simulink model "sm_amrPioneer3DX_path_follow"  (R2025a)
settings: Solver=ode23t  StartTime=0.0  StopTime=35  RelTol=1e-3  AbsTol=1e-4
PostLoadFcn:
  | waypoints = [0 0; 4 2; 3 7; -3 6];
  | target_vel = 0.5;
  | lookahead_d = 2;
  | max_yaw_rate = 1;
StopFcn:
  | %robotPoses = out.yout{1}.Values.Data;
  | 
  | %figure(99);
  | %plot(waypoints(:,1), waypoints(:,2), 'k-x');
  | %hold all
  | %plot(robotPoses(:,1), robotPoses(:,2));
  | %title('XY Waypoint Tracking');
undefined symbols (not defined in the file or in its folder): X, Y, Z
libraries: sm_lib x100, nesl_utility x11, robotalgslib x1, simulink x1
(part 1 of 3)
CloseFcn:
  | try,close(h1_sm_amrPioneer3DX_path_follow),end
  | clear h1_sm_amrPioneer3DX_path_follow
  | try,close(h2_sm_amrPioneer3DX_path_follow),end
  | clear h2_sm_amrPioneer3DX_path_follow
  | try,close(h3_sm_amrPioneer3DX_path_follow),end
  | clear h3_sm_amrPioneer3DX_path_follow
  | try,close(h4_sm_amrPioneer3DX_path_follow),end
  | clear h4_sm_amrPioneer3DX_path_follow
Description:
  | Differential Drive Robot Following a Path
  | Copyright 2021-2025 The MathWorks, Inc.
settings Model: PacingRate=0.011000  Creator=The MathWorks, Inc.  LastModifiedBy=smiller
settings SolverCC: AlgebraicLoopSolver=TrustRegion
settings DataIOCC: MaxDataPoints=10000  SaveOutput=off  ReturnWorkspaceOutputs=off  SignalLoggingName=logsout_sm_amrPioneer3DX_path_follow
settings OptimizationCC: ReuseModelBlockBuffer=off
settings DebuggingCC: UnconnectedInputMsg=warning  UnconnectedOutputMsg=warning  UnconnectedLineMsg=warning  SymbolicDimsDataTypeCodeGenerationDiagnostic=none
settings ModelReferenceCC: EnableRefExpFcnMdlSchedulingChecks=on
settings RTWCC: GPUComputeCapability=3.5  DLArmComputeVersion=19.05
settings SimscapeCC: SimscapeLogType=all  SimscapeLogSimulationStatistics=on  SimscapeLogName=simlog_sm_amrPioneer3DX_path_follow  SimscapeLogDataHistory=10000.0
settings DiagnosticsConfigSet: SimMechanicsConflictingReferenceFrames=none  SimMechanicsRigidlyBoundBlock=none
settings ExplorerConfigSet: InternalSimMechanicsExplorerSettings="<ExplorerConfiguration><canonicalview>default</canonicalview><AnimationSetting><BasePlaybackSpeed>1.0</BasePlaybackSpeed><PlaybackSpeedFactor>4.0</PlaybackSpeedFactor></AnimationSetting><TilePanel><TileInfo><Tiles Columns=\"2\" Count=\"2\" Rows=\"1\"><Column Weight=\"0.5\"/><Column Weight=\"0.5\"/><Row Weight=\"1\"/><Tile Height=\"1\" Width=\"1\" X=\"0\" Y=\"0\"/><Tile Height=\"1\" Width=\"1\" X=\"1\" Y=\"0\"/></Tiles></TileInfo><SceneInfo><SceneViewer><BGColor><R>1</R><G>1</G><B>1</B></BGColor><Camera><DoPerspective>on</DoPerspective><Position><X>-0.845000000000000084</X><Y>0</Y><Z>0.44900000000000001</Z></Position><Center><X>0.139807753012207936</X><Y>0</Y><Z>0.275351822333069651</Z></Center><Up><X>0.173648177666930359</X><Y>0</Y><Z>0.98480775301220802</Z></Up><ViewLimDist>1</ViewLimDist><YLim>0.466307658154998583</YLim><XLim>0.535867364067622698</XLim></Camera></SceneViewer><SceneViewer><BGColor><R>1</R><G>1</G><B>1</B></BGColor><Camera><DoPerspective>off</DoPerspective><Position><X>0.52473266601562496</X><Y>3.27863929130782239</Y><Z>4.85881988452804414</Z></Position><Center><X>0.52473266601562496</X><Y>3.27863929130782239</Y><Z>0.120798183548071592</Z></Center><Up><X>0</X><Y>1</Y><Z>-0</Z></Up><ViewLimDist>1</ViewLimDist><YLim>3.89199849605560333</YLim><XLim>4.47257285734566512</XLim></Camera></SceneViewer></SceneInfo></TilePanel><MechEditorPanel><Cameras><Camera><Id>Camera1</Id><Value><Name>Track_Rear</Name><NativeCamera><PositionTrackingFeature>Robot.Camera.Reference_Frame_Camera_Rear.R</PositionTrackingFeature><CenterTrackingFeature>Robot.Camera.Reference_Frame_Camera_Rear.R</CenterTrackingFeature><UpVectorTrackingFeature>Robot.Camera.Reference_Frame_Camera_Rear.R</UpVectorTrackingFeature><CenterTrackingOrigin>off</CenterTrackingOrigin><CenterTrackingDirection>+X</CenterTrackingDirection><UpVectorTrackingDirection>+Z</UpVectorTrackingDirection></NativeCamera></Value></Camera><Camera><Id>Camera2</Id><Value><Name>Track_Left</Name><NativeCamera><PositionTrackingFeature>Robot.Camera.Reference_Frame_Camera_Left.R</PositionTrackingFeature><CenterTrackingFeature>Robot.Camera.Reference_Frame_Camera_Left.R</CenterTrackingFeature><UpVectorTrackingFeature>Robot.Camera.Reference_Frame_Camera_Left.R</UpVectorTrackingFeature><CenterTrackingOrigin>off</CenterTrackingOrigin><CenterTrackingDirection>+X</CenterTrackingDirection><UpVectorTrackingDirection>+Z</UpVectorTrackingDirection></NativeCamera></Value></Camera></Cameras><GfxPanelCameraMap><MapElement CameraMLId=\"Camera1\" GfxPanelIndex=\"0\"/></GfxPanelCameraMap><VideoCreator><PlaybackSpeedRatio>1.0</PlaybackSpeedRatio><FrameRate>30</FrameRate><VideoFormat>Motion JPEG AVI</VideoFormat><FrameSize>auto</FrameSize></VideoCreator></MechEditorPanel></ExplorerConfiguration>"

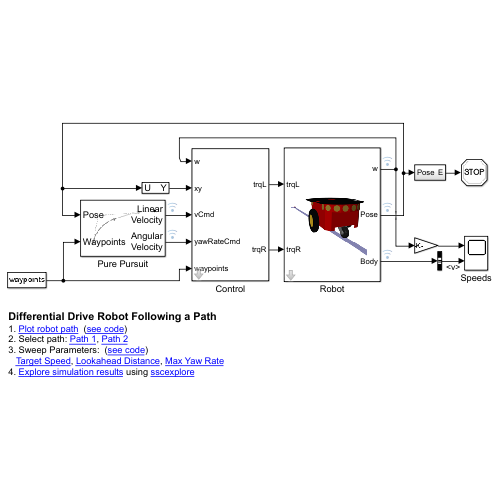
[thumbnail: Simulink's stored preview of the top-level diagram]
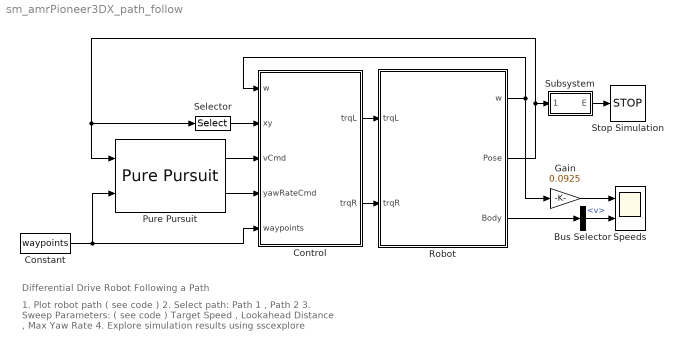
== system sm_amrPioneer3DX_path_follow ==
  note: Differential Drive Robot Following a Path
  note: 1. Plot robot path ( see code )
      | 2. Select path: Path 1 , Path 2
      | 3. Sweep Parameters: ( see code )
      | Target Speed , Lookahead Distance , Max Yaw Rate
      | 4. Explore simulation results using sscexplore
  Bus Selector : BusSelector  OutputSignals=v
  Constant : Constant  Value=waypoints
  Control : Subsystem  mask(Control for Differential Drive Robot){xTrack=0.3, rWheel=0.0925, xSlow=0.5, xStop=0.1, kp=0.8}
      mask prompts: xTrack "Robot Drive Wheel Radius (m)"; rWheel "Robot Track Width (m)"; xSlow "Distance from end to slow (m)"; xStop "Distance from end to stop (m)"; kp "Controller Proportional Gain"
      mask help: Determines torque commands for wheels based on target speed and target yaw rate of robot. As robot approaches final waypoint, speed is ramped down to 0.
  Gain : Gain  Gain=0.0925
  Pure Pursuit : robotalgslib/Pure Pursuit  DesiredLinearVelocityPort=off  DesiredLinearVelocity=target_vel  MaxAngularVelocity=max_yaw_rate  LookaheadDistancePort=off  LookaheadDistance=lookahead_d  TargetDirPort=off  SimulateUsing=Code generation
  Robot : Subsystem  mask(Differential Drive Robot){kWheel=1e4, dWheel=1e3, xtrWheel=1e-3, muk=0.9, mud=0.8, vth=1e-3, checkbox_start=on, waypoint_list=waypoints, init_xy_user=[0 0], init_orient_user=0, clr_contact_sphere=[0 1 0], opc_contact_sphere=0}
      mask prompts: kWheel "Stiffness (N/m)"; dWheel "Damping (N/(m/s))"; xtrWheel "Transition Region Width (m)"; muk "Static Friction Coefficient"; mud "Dynamic Friction Coefficient"; vth "Critical Velocity (m/s)"; checkbox_start "Start at first waypoint"; waypoint_list "Waypoints [xy] (m)"; init_xy_user "Initial Position [x y] (m)"; init_orient_user "Initial Orientation  (0 = +x) (deg)"; clr_contact_sphere "Color Contact Spheres [RGB]"; opc_contact_sphere "Opacity Contact Spheres"
      mask help: Set contact, friction, and initial pose for robot.
      mask init:
      | if (strcmp(get_param(gcb,'checkbox_start'),'on'))
      |   init_orient = atan2(waypoint_list(2,2)-waypoint_list(1,2),waypoint_list(2,1)-waypoint_list(1,1))*180/pi;
      |   init_xy = waypoint_list(1,:);
      | else
      |   init_xy     = init_xy_user;
      |   init_orient = init_orient_user;
      | end
      mask Callback checkbox_start:
      | maskObj = Simulink.Mask.get(gcb);
      | wpl_h = maskObj.getParameter('waypoint_list');
      | ixy_h = maskObj.getParameter('init_xy_user');
      | ior_h = maskObj.getParameter('init_orient_user');
      | if (strcmp(get_param(gcb,'checkbox_start'),'on'))
      |     wpl_h.Visible = 'on';
      |     ixy_h.Visible = 'off';
      |     ior_h.Visible = 'off';
      | else
      |     wpl_h.Visible = 'off';
      |     ixy_h.Visible = 'on';
      |     ior_h.Visible = 'on';
      | end
      mask DialogControl grp_whl_contact Prompt: Wheel Contact
      mask Display: image('sm_amrPioneer3DX_path_follow_robot.png')
  Selector : Selector  InputPortWidth=3  IndexOptions=Index vector (dialog)  Indices=[1 2]  OutputSizes=1
  Speeds : Scope  NumInputPorts=2
      settings: ActiveDisplayYMinimum=-0.11386  ActiveDisplayYMaximum=1.02475
  Stop Simulation : Stop
  Subsystem : Subsystem
  wires:
  Constant/1 -> Pure Pursuit/2, Control/5(waypoints)
  Robot/1(w) -> Gain/1, Control/1(w)
  Robot/2(Pose) -> Selector/1, Pure Pursuit/1, Subsystem/1(Pose)
  Gain/1 -> Speeds/1
  Robot/3(Body) -> Bus Selector/1
  Pure Pursuit/1 -> Control/3(vCmd)
  Pure Pursuit/2 -> Control/4(yawRateCmd)
  Control/1(trqL) -> Robot/1(trqL)
  Control/2(trqR) -> Robot/2(trqR)
  Selector/1 -> Control/2(xy)
  Subsystem/1(E) -> Stop Simulation/1
  Bus Selector/1 -> Speeds/2  "<v>"

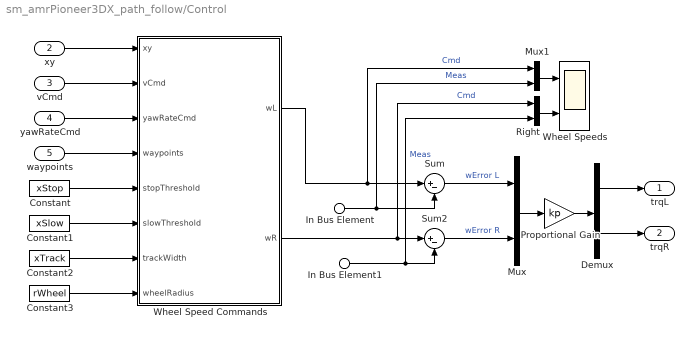
== system sm_amrPioneer3DX_path_follow/Control ==
  In Bus Element : Inport  PortName=w  Element=L
  In Bus Element1 : Inport  PortName=w  Element=R
  xy : Inport  Port=2
  vCmd : Inport  Port=3
  yawRateCmd : Inport  Port=4
  waypoints : Inport  Port=5
  Constant : Constant  Value=xStop
  Constant1 : Constant  Value=xSlow
  Constant2 : Constant  Value=xTrack
  Constant3 : Constant  Value=rWheel
  Demux : Demux  Outputs=2
  Mux : Mux  Inputs=2
  Mux1 : Mux  Inputs=2
  Proportional Gain : Gain  Gain=kp
  Right : Mux  Inputs=2
  Sum : Sum  Inputs=|+-
  Sum2 : Sum  Inputs=|+-
  Wheel Speed Commands : MATLAB Function  TreatAsAtomicUnit=on
  Wheel Speeds : Scope  NumInputPorts=2
      settings: Title=Left Wheel  ActiveDisplayYMinimum=-0.75851  ActiveDisplayYMaximum=6.82662  DataLoggingVariableName=ScopeData2
  trqL : Outport
  trqR : Outport  Port=2
  wires:
  Demux/1 -> trqL/1
  yawRateCmd/1 -> Wheel Speed Commands/3(yawRateCmd)
  xy/1 -> Wheel Speed Commands/1(xy)
  vCmd/1 -> Wheel Speed Commands/2(vCmd)
  Demux/2 -> trqR/1
  waypoints/1 -> Wheel Speed Commands/4(waypoints)
  Constant/1 -> Wheel Speed Commands/5(stopThreshold)
  Constant1/1 -> Wheel Speed Commands/6(slowThreshold)
  Constant2/1 -> Wheel Speed Commands/7(trackWidth)
  Constant3/1 -> Wheel Speed Commands/8(wheelRadius)
  Wheel Speed Commands/1(wL) -> Mux1/1, Sum/1  "Cmd"
  Wheel Speed Commands/2(wR) -> Right/1, Sum2/1  "Cmd"
  Sum2/1 -> Mux/2  "wError R"
  In Bus Element1/1 -> Sum2/2, Right/2  "Meas"
  In Bus Element/1 -> Mux1/2, Sum/2  "Meas"
  Mux/1 -> Proportional Gain/1
  Proportional Gain/1 -> Demux/1
  Sum/1 -> Mux/1  "wError L"
  Mux1/1 -> Wheel Speeds/1
  Right/1 -> Wheel Speeds/2

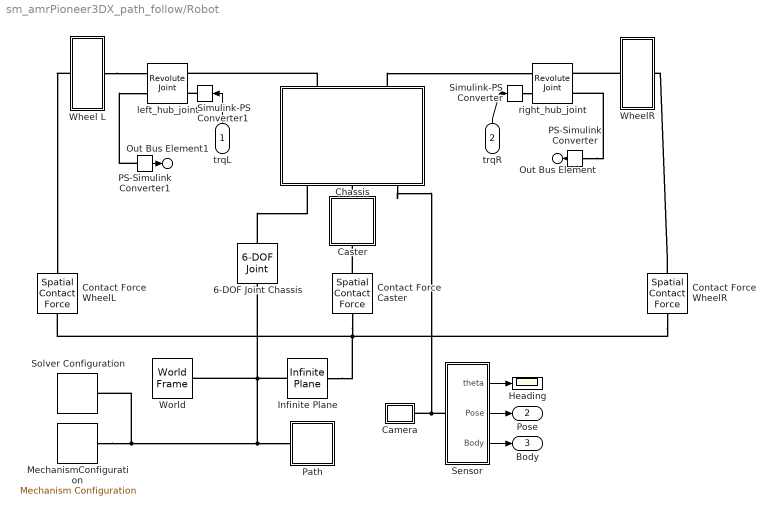
== system sm_amrPioneer3DX_path_follow/Robot ==
  trqL : Inport
  trqR : Inport  Port=2
  6-DOF Joint Chassis : sm_lib/Joints/6-DOF Joint  JointMode=Normal  CompositeWrenchDir=FollowerOnBase  CompositeWrenchFrame=BaseFrame  SenseConstraintForce=off  SenseConstraintTorque=off  SenseTotalForce=off  SenseTotalTorque=off  PxPositionTargetSpecify=on  PxPositionTargetPriority=High  PxPositionTargetValue=init_xy(1)  PxPositionTargetValueUnits=m  PxVelocityTargetSpecify=off  PxVelocityTargetPriority=High  PxVelocityTargetValue=0  PxVelocityTargetValueUnits=m/s  PxEquilibriumPosition=0  PxEquilibriumPositionUnits=m  PxSpringStiffness=0  PxSpringStiffnessUnits=N/m  PxDampingCoefficient=0  PxDampingCoefficientUnits=N/(m/s)  PxLowerLimitSpecify=off  PxLowerLimitBound=-1  PxLowerLimitBoundUnits=m  PxLowerLimitStiffness=1e6  PxLowerLimitStiffnessUnits=N/m  PxLowerLimitDamping=1e3  PxLowerLimitDampingUnits=N/(m/s)  PxLowerLimitTransitionRegionWidth=1e-4  PxLowerLimitTransitionRegionWidthUnits=m  PxUpperLimitSpecify=off  PxUpperLimitBound=1  PxUpperLimitBoundUnits=m  PxUpperLimitStiffness=1e6  PxUpperLimitStiffnessUnits=N/m  PxUpperLimitDamping=1e3  PxUpperLimitDampingUnits=N/(m/s)  PxUpperLimitTransitionRegionWidth=1e-4  PxUpperLimitTransitionRegionWidthUnits=m  PxTorqueActuationMode=NoTorque  PxMotionActuationMode=ComputedMotion  PxSensePosition=off  PxSenseVelocity=off  PxSenseAcceleration=off  PxSenseTorqueForce=off  PxSenseLowerLimitTorqueForce=off  PxSenseUpperLimitTorqueForce=off  PyPositionTargetSpecify=on  PyPositionTargetPriority=High  PyPositionTargetValue=init_xy(2)  PyPositionTargetValueUnits=m  PyVelocityTargetSpecify=off  PyVelocityTargetPriority=High  PyVelocityTargetValue=0  PyVelocityTargetValueUnits=m/s  PyEquilibriumPosition=0  PyEquilibriumPositionUnits=m  PySpringStiffness=0  PySpringStiffnessUnits=N/m  PyDampingCoefficient=0  PyDampingCoefficientUnits=N/(m/s)  PyLowerLimitSpecify=off  PyLowerLimitBound=-1  PyLowerLimitBoundUnits=m  PyLowerLimitStiffness=1e6  PyLowerLimitStiffnessUnits=N/m  PyLowerLimitDamping=1e3  PyLowerLimitDampingUnits=N/(m/s)  PyLowerLimitTransitionRegionWidth=1e-4  PyLowerLimitTransitionRegionWidthUnits=m  PyUpperLimitSpecify=off  PyUpperLimitBound=1  PyUpperLimitBoundUnits=m  PyUpperLimitStiffness=1e6  PyUpperLimitStiffnessUnits=N/m  PyUpperLimitDamping=1e3  PyUpperLimitDampingUnits=N/(m/s)  PyUpperLimitTransitionRegionWidth=1e-4  PyUpperLimitTransitionRegionWidthUnits=m  PyTorqueActuationMode=NoTorque  PyMotionActuationMode=ComputedMotion  PySensePosition=off  PySenseVelocity=off  PySenseAcceleration=off  PySenseTorqueForce=off  PySenseLowerLimitTorqueForce=off  PySenseUpperLimitTorqueForce=off  PzPositionTargetSpecify=on  PzPositionTargetPriority=High  PzPositionTargetValue=0.015  PzPositionTargetValueUnits=m  PzVelocityTargetSpecify=off  PzVelocityTargetPriority=High  PzVelocityTargetValue=0  PzVelocityTargetValueUnits=m/s  PzEquilibriumPosition=0  PzEquilibriumPositionUnits=m  PzSpringStiffness=0  PzSpringStiffnessUnits=N/m  PzDampingCoefficient=0  PzDampingCoefficientUnits=N/(m/s)  PzLowerLimitSpecify=off  PzLowerLimitBound=-1  PzLowerLimitBoundUnits=m  PzLowerLimitStiffness=1e6  PzLowerLimitStiffnessUnits=N/m  PzLowerLimitDamping=1e3  PzLowerLimitDampingUnits=N/(m/s)  PzLowerLimitTransitionRegionWidth=1e-4  PzLowerLimitTransitionRegionWidthUnits=m  PzUpperLimitSpecify=off  PzUpperLimitBound=1  PzUpperLimitBoundUnits=m  PzUpperLimitStiffness=1e6  PzUpperLimitStiffnessUnits=N/m  PzUpperLimitDamping=1e3  PzUpperLimitDampingUnits=N/(m/s)  PzUpperLimitTransitionRegionWidth=1e-4  PzUpperLimitTransitionRegionWidthUnits=m  PzTorqueActuationMode=NoTorque  PzMotionActuationMode=ComputedMotion  PzSensePosition=off  PzSenseVelocity=off  PzSenseAcceleration=off  PzSenseTorqueForce=off  PzSenseLowerLimitTorqueForce=off  PzSenseUpperLimitTorqueForce=off  SphPositionTargetSpecify=on  SphPositionTargetPriority=High  SphPositionTargetRotationMethod=StandardAxis  SphPositionTargetFollAlignAxisA=+X  SphPositionTargetBaseAlignAxisA=+Y  SphPositionTargetFollAlignAxisB=+Y  SphPositionTargetBaseAlignAxisB=+Z  SphPositionTargetRotationStandardAxis=+Z  SphPositionTargetRotationAngle=init_orient  SphPositionTargetRotationAngleUnits=deg  SphPositionTargetRotationArbitraryAxis=[0 0 1]  SphPositionTargetRotationSequenceAxes=FollowerAxes  SphPositionTargetRotationSequence=XYX  SphPositionTargetRotationSequenceAngles=[0 0 0]  SphPositionTargetRotationSequenceAnglesUnits=deg  SphPositionTargetRotationMatrix=[1 0 0; 0 1 0; 0 0 1]  SphPositionTargetQuaternion=[1 0 0 0]  SphVelocityTargetSpecify=off  SphVelocityTargetPriority=High  SphVelocityTargetValue=[0 0 0]  SphVelocityTargetValueUnits=deg/s  SphVelocityTargetInFollowerFrame=on  SphEqPosRotationMethod=None  SphEqPosFollAlignAxisA=+X  SphEqPosBaseAlignAxisA=+Y  SphEqPosFollAlignAxisB=+Y  SphEqPosBaseAlignAxisB=+Z  SphEqPosRotationStandardAxis=+Z  SphEqPosRotationAngle=0.0  SphEqPosRotationAngleUnits=deg  SphEqPosRotationArbitraryAxis=[0 0 1]  SphEqPosRotationSequenceAxes=FollowerAxes  SphEqPosRotationSequence=XYX  SphEqPosRotationSequenceAngles=[0 0 0]  SphEqPosRotationSequenceAnglesUnits=deg  SphEqPosRotationMatrix=[1 0 0; 0 1 0; 0 0 1]  SphEqPosQuaternion=[1 0 0 0]  SphSpringStiffness=0  SphSpringStiffnessUnits=N*m/deg  SphDampingCoefficient=0  SphDampingCoefficientUnits=N*m/(deg/s)  SphLowerLimitSpecify=off  SphLowerLimitBound=15  SphLowerLimitBoundUnits=deg  SphLowerLimitStiffness=1e4  SphLowerLimitStiffnessUnits=N*m/deg  SphLowerLimitDamping=10  SphLowerLimitDampingUnits=N*m/(deg/s)  SphLowerLimitTransitionRegionWidth=0.1  SphLowerLimitTransitionRegionWidthUnits=deg  SphUpperLimitSpecify=off  SphUpperLimitBound=45  SphUpperLimitBoundUnits=deg  SphUpperLimitStiffness=1e4  SphUpperLimitStiffnessUnits=N*m/deg  SphUpperLimitDamping=10  SphUpperLimitDampingUnits=N*m/(deg/s)  SphUpperLimitTransitionRegionWidth=0.1  SphUpperLimitTransitionRegionWidthUnits=deg  SphTorqueActuationMode=NoTorque  SphActuateTorqueX=off  SphActuateTorqueY=off  SphActuateTorqueZ=off  SphActuateTorque=off  SphActuationFrame=BaseFrame  SphSensePosition=off  SphSenseVelocityX=off  SphSenseVelocityY=off  SphSenseVelocityZ=off  SphSenseVelocity=off  SphSenseAccelerationX=off  SphSenseAccelerationY=off  SphSenseAccelerationZ=off  SphSenseAcceleration=off  SphSenseLowerLimitTorqueMag=off  SphSenseUpperLimitTorqueMag=off  SphSensingFrame=BaseFrame
  Camera : Subsystem
  Caster : Subsystem
  Chassis : Subsystem
  Contact Force Caster : sm_lib/Forces and Torques/Spatial Contact Force  SenseSeparationDistance=off  NormalForceType=SmoothSpringDamper  NormalStiffness=kWheel  NormalStiffnessUnits=N/m  NormalDamping=dWheel  NormalDampingUnits=N/(m/s)  NormalTransitionRegionWidth=xtrWheel  NormalTransitionRegionWidthUnits=m  FrictionType=SmoothStickSlip  CoefficientOfStaticFriction=muk  CoefficientOfDynamicFriction=mud  FrictionalCriticalVelocity=vth  FrictionalCriticalVelocityUnits=m/s  SenseContactSignal=off  SensePenetrationDepth=off  SenseNormalVelocity=off  SenseTangentialVelocity=off  SensingForceTorqueDirection=BaseOnFollower  SensingForceTorqueResolutionFrame=ContactFrame  SenseNormalForce=off  SenseNormalForceMagnitude=off  SenseNormalTorque=off  SenseFrictionalForce=off  SenseFrictionalForceMagnitude=off  SenseFrictionalTorque=off  SenseTotalForce=off  SenseTotalTorque=off  SenseContactBaseRotation=off  SenseContactBaseTranslation=off  SenseContactFollowerRotation=off  SenseContactFollowerTranslation=off  ZeroCrossDetectContactStartAndEnd=off
  Contact Force WheelL : sm_lib/Forces and Torques/Spatial Contact Force  SenseSeparationDistance=off  NormalForceType=SmoothSpringDamper  NormalStiffness=kWheel  NormalStiffnessUnits=N/m  NormalDamping=dWheel  NormalDampingUnits=N/(m/s)  NormalTransitionRegionWidth=xtrWheel  NormalTransitionRegionWidthUnits=m  FrictionType=SmoothStickSlip  CoefficientOfStaticFriction=muk  CoefficientOfDynamicFriction=mud  FrictionalCriticalVelocity=vth  FrictionalCriticalVelocityUnits=m/s  SenseContactSignal=off  SensePenetrationDepth=off  SenseNormalVelocity=off  SenseTangentialVelocity=off  SensingForceTorqueDirection=BaseOnFollower  SensingForceTorqueResolutionFrame=ContactFrame  SenseNormalForce=off  SenseNormalForceMagnitude=off  SenseNormalTorque=off  SenseFrictionalForce=off  SenseFrictionalForceMagnitude=off  SenseFrictionalTorque=off  SenseTotalForce=off  SenseTotalTorque=off  SenseContactBaseRotation=off  SenseContactBaseTranslation=off  SenseContactFollowerRotation=off  SenseContactFollowerTranslation=off  ZeroCrossDetectContactStartAndEnd=off
  Contact Force WheelR : sm_lib/Forces and Torques/Spatial Contact Force  SenseSeparationDistance=off  NormalForceType=SmoothSpringDamper  NormalStiffness=kWheel  NormalStiffnessUnits=N/m  NormalDamping=dWheel  NormalDampingUnits=N/(m/s)  NormalTransitionRegionWidth=xtrWheel  NormalTransitionRegionWidthUnits=m  FrictionType=SmoothStickSlip  CoefficientOfStaticFriction=muk  CoefficientOfDynamicFriction=mud  FrictionalCriticalVelocity=vth  FrictionalCriticalVelocityUnits=m/s  SenseContactSignal=off  SensePenetrationDepth=off  SenseNormalVelocity=off  SenseTangentialVelocity=off  SensingForceTorqueDirection=BaseOnFollower  SensingForceTorqueResolutionFrame=ContactFrame  SenseNormalForce=off  SenseNormalForceMagnitude=off  SenseNormalTorque=off  SenseFrictionalForce=off  SenseFrictionalForceMagnitude=off  SenseFrictionalTorque=off  SenseTotalForce=off  SenseTotalTorque=off  SenseContactBaseRotation=off  SenseContactBaseTranslation=off  SenseContactFollowerRotation=off  SenseContactFollowerTranslation=off  ZeroCrossDetectContactStartAndEnd=off
  Heading : Scope
      settings: ActiveDisplayYMinimum=-3.92553  ActiveDisplayYMaximum=3.92324
  Infinite Plane : sm_lib/Curves and Surfaces/Infinite Plane  GraphicType=Rectangle  GraphicPlaneWidth=1  GraphicPlaneWidthUnits=m  GraphicPlaneHeight=1  GraphicPlaneHeightUnits=m  GraphicVisPropType=SimpleVisualProperties  GraphicDiffuseColor=[0.5 0.5 0.5]  GraphicOpacity=0.25  GraphicSpecularColor=[0.5 0.5 0.5 1.0]  GraphicAmbientColor=[0.15 0.15 0.15 1.0]  GraphicEmissiveColor=[0.0 0.0 0.0 1.0]  GraphicShininess=75
  MechanismConfiguration : sm_lib/Utilities/Mechanism Configuration  UniformGravity=Constant  GravityVector=[0 0 -9.80665]  GravityVectorUnits=m/s^2  LinearizationDelta=0.001  JointModeTransitionNonlinearIterations=2
  PS-Simulink Converter : nesl_utility/PS-Simulink Converter  PhysicalDomain=network_engine_domain  SubClassName=ps_output  LeftPortType=input  RightPortType=output  PseudoPeriodic=off  Frequencies=[]  VectorFormat=1-D array  Unit=inherit  AffineConversion=off
  PS-Simulink Converter1 : nesl_utility/PS-Simulink Converter  PhysicalDomain=network_engine_domain  SubClassName=ps_output  LeftPortType=input  RightPortType=output  PseudoPeriodic=off  Frequencies=[]  VectorFormat=1-D array  Unit=inherit  AffineConversion=off
  Path : Subsystem  mask(Visualize Path of Waypoints){waypoints=waypoints, path_width=0.03, path_depth=0.01, clr_path=[0.6 0.6 1], opc_path=0.5, pt_rad=2e-2, pt_clr=[0.6353 0.07843 0.1843], pt_opc=0.8}
      mask prompts: waypoints "Waypoints [x y] (m)"; path_width "Path Width (m)"; path_depth "Path Depth (m)"; clr_path "Path Color [RGB]"; opc_path "Path Opacity (0-1)"; pt_rad "Waypoints Radius"; pt_clr "Waypoints Color [RGB]"; pt_opc "Waypoints Opacity (0-1)"
      mask help: Visualize path of waypoints using point cloud for points and extrusion for path. Path must not cross itself.
      mask init:
      | xy_data = Extr_Data_Waypoints(waypoints,path_width);
  Sensor : Subsystem
  Simulink-PS Converter : nesl_utility/Simulink-PS Converter  PhysicalDomain=network_engine_domain  SubClassName=ps_input  LeftPortType=input  RightPortType=output  PseudoPeriodic=off  Frequencies=[]  NoiseDistribution=none  NoiseParameters=[]  Unit=1  AffineConversion=off  FilteringAndDerivatives=provide  SimscapeFilterOrder=1  InputFilterTimeConstant=0.001  UdotUserProvided=0
  Simulink-PS Converter1 : nesl_utility/Simulink-PS Converter  PhysicalDomain=network_engine_domain  SubClassName=ps_input  LeftPortType=input  RightPortType=output  PseudoPeriodic=off  Frequencies=[]  NoiseDistribution=none  NoiseParameters=[]  Unit=1  AffineConversion=off  FilteringAndDerivatives=provide  SimscapeFilterOrder=1  InputFilterTimeConstant=0.001  UdotUserProvided=0
  Solver Configuration : nesl_utility/Solver Configuration  PhysicalDomain=network_engine_domain  SubClassName=solver  LeftPortType=input  RightPortType=generic  Tones=[]  Harmonics=[]  SimulateNoise=off  Profile=off  UseLocalSampling=off  EnableSwitchedLinearOptims=on  FrequencyDomain=off  UseCCode=off  RelTol=0.001  AbsTol=1e-06  MinStep=1e-09  ToWorkspace=off  RevertToSquareIcSolve=off  NumHomotopyIterations=100  PhasorMode=off  PhasorModeNumHarmonics=1  ConsistencySolver=NEWTON_FTOL  IndexReductionMethod=DerivativeReplacement  DoDC=off  ResidualTolerance=1e-09  ConsistencyTolSource=GLOBAL  ConsistencyAbsTol=0.001  ConsistencyRelTol=0.001  ConsistencyTolFactor=0.001  UseLocalSolver=off  LocalSolverChoice=NE_BACKWARD_EULER_ADVANCER  ResolveIndetEquations=on  FunctionEvalNumThread=1  LocalSolverSampleTime=0.001  DoFixedCost=off  MaxNonlinIter=3  MaxModeIter=2  ComputeImpulses=off  ImpulseIterations=2  LinearAlgebra=auto  LinearAlgebraNumThread=0  EquationFormulation=NE_TIME_EF  DelaysMemoryBudget=1024  AutomaticFiltering=on  FilteringTimeConstant=0.001  PartitionStorageMethod=AS_NEEDED  PartitionMemoryBudget=1024  PartitionMethod=ROBUST  MultibodyUseLocalSolver=off  MultibodyLocalSolverChoice=ODE1  MultibodyLocalSolverSampleTime=0.001
  Wheel L : Subsystem
  WheelR : Subsystem
  World : sm_lib/Frames and Transforms/World Frame
  left_hub_joint : sm_lib/Joints/Revolute Joint  JointMode=Normal  CompositeWrenchDir=FollowerOnBase  CompositeWrenchFrame=BaseFrame  SenseConstraintForce=off  SenseConstraintTorque=off  SenseTotalForce=off  SenseTotalTorque=off  PositionTargetSpecify=off  PositionTargetPriority=High  PositionTargetValue=0  PositionTargetValueUnits=deg  VelocityTargetSpecify=off  VelocityTargetPriority=High  VelocityTargetValue=0  VelocityTargetValueUnits=deg/s  EquilibriumPosition=0  EquilibriumPositionUnits=deg  SpringStiffness=0  SpringStiffnessUnits=N*m/deg  DampingCoefficient=0  DampingCoefficientUnits=m^2*kg/s/rad  LowerLimitSpecify=off  LowerLimitBound=-90  LowerLimitBoundUnits=deg  LowerLimitStiffness=1e4  LowerLimitStiffnessUnits=N*m/deg  LowerLimitDamping=10  LowerLimitDampingUnits=N*m/(deg/s)  LowerLimitTransitionRegionWidth=0.1  LowerLimitTransitionRegionWidthUnits=deg  UpperLimitSpecify=off  UpperLimitBound=90  UpperLimitBoundUnits=deg  UpperLimitStiffness=1e4  UpperLimitStiffnessUnits=N*m/deg  UpperLimitDamping=10  UpperLimitDampingUnits=N*m/(deg/s)  UpperLimitTransitionRegionWidth=0.1  UpperLimitTransitionRegionWidthUnits=deg  TorqueActuationMode=InputTorque  MotionActuationMode=ComputedMotion  SensePosition=off  SenseVelocity=on  SenseAcceleration=off  SenseTorqueForce=off  SenseLowerLimitTorqueForce=off  SenseUpperLimitTorqueForce=off
  right_hub_joint : sm_lib/Joints/Revolute Joint  JointMode=Normal  CompositeWrenchDir=FollowerOnBase  CompositeWrenchFrame=BaseFrame  SenseConstraintForce=off  SenseConstraintTorque=off  SenseTotalForce=off  SenseTotalTorque=off  PositionTargetSpecify=off  PositionTargetPriority=High  PositionTargetValue=0  PositionTargetValueUnits=deg  VelocityTargetSpecify=off  VelocityTargetPriority=High  VelocityTargetValue=0  VelocityTargetValueUnits=deg/s  EquilibriumPosition=0  EquilibriumPositionUnits=deg  SpringStiffness=0  SpringStiffnessUnits=N*m/deg  DampingCoefficient=0  DampingCoefficientUnits=m^2*kg/s/rad  LowerLimitSpecify=off  LowerLimitBound=-90  LowerLimitBoundUnits=deg  LowerLimitStiffness=1e4  LowerLimitStiffnessUnits=N*m/deg  LowerLimitDamping=10  LowerLimitDampingUnits=N*m/(deg/s)  LowerLimitTransitionRegionWidth=0.1  LowerLimitTransitionRegionWidthUnits=deg  UpperLimitSpecify=off  UpperLimitBound=90  UpperLimitBoundUnits=deg  UpperLimitStiffness=1e4  UpperLimitStiffnessUnits=N*m/deg  UpperLimitDamping=10  UpperLimitDampingUnits=N*m/(deg/s)  UpperLimitTransitionRegionWidth=0.1  UpperLimitTransitionRegionWidthUnits=deg  TorqueActuationMode=InputTorque  MotionActuationMode=ComputedMotion  SensePosition=off  SenseVelocity=on  SenseAcceleration=off  SenseTorqueForce=off  SenseLowerLimitTorqueForce=off  SenseUpperLimitTorqueForce=off
  Out Bus Element : Outport  PortName=w  Element=R
  Out Bus Element1 : Outport  PortName=w  Element=L
  Pose : Outport  Port=2
  Body : Outport  Port=3
  wires:
  PS-Simulink Converter1/1 -> Out Bus Element1/1
  PS-Simulink Converter/1 -> Out Bus Element/1
  trqR/1 -> Simulink-PS Converter/1
  trqL/1 -> Simulink-PS Converter1/1
  Sensor/3(Body) -> Body/1
  Sensor/1(theta) -> Heading/1
  Sensor/2(Pose) -> Pose/1
  connections:
  Infinite Plane/RConn1 -- Contact Force WheelR/LConn1 -- Contact Force Caster/LConn1 -- Contact Force WheelL/LConn1
  MechanismConfiguration/RConn1 -- Solver Configuration/RConn1 -- World/RConn1 -- Infinite Plane/LConn1 -- 6-DOF Joint Chassis/LConn1 -- Path/LConn1
  Simulink-PS Converter1/RConn1 -- left_hub_joint/LConn2
  PS-Simulink Converter/LConn1 -- right_hub_joint/RConn2
  PS-Simulink Converter1/LConn1 -- left_hub_joint/RConn2
  Simulink-PS Converter/RConn1 -- right_hub_joint/LConn2
  Chassis/RConn2 -- right_hub_joint/LConn1
  Chassis/RConn1 -- left_hub_joint/LConn1
  6-DOF Joint Chassis/RConn1 -- Chassis/LConn1
  Caster/LConn1 -- Chassis/LConn2
  Contact Force Caster/RConn1 -- Caster/RConn1
  WheelR/LConn1 -- right_hub_joint/RConn1
  Contact Force WheelR/RConn1 -- WheelR/RConn1
  Wheel L/RConn1 -- left_hub_joint/RConn1
  Wheel L/LConn1 -- Contact Force WheelL/RConn1
  Sensor/LConn1 -- Chassis/LConn3 -- Camera/LConn1

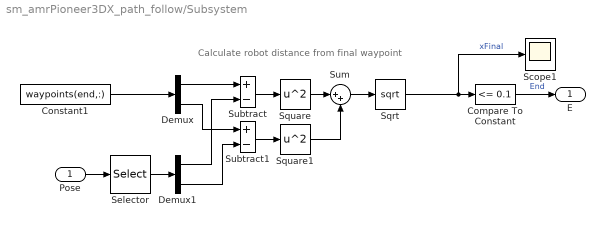
== system sm_amrPioneer3DX_path_follow/Subsystem ==
  note: Calculate robot distance
      | from final waypoint
  Pose : Inport
  Compare To Constant : simulink/Logic and Bit Operations/Compare To Constant  relop=<=  const=0.1  OutDataTypeStr=boolean
  Constant1 : Constant  Value=waypoints(end,:)
  Demux : Demux  Outputs=2
  Demux1 : Demux  Outputs=2
  Scope1 : Scope
      settings: ActiveDisplayYMinimum=-0.84679  ActiveDisplayYMaximum=8.62109  DataLoggingVariableName=ScopeData2
  Selector : Selector  InputPortWidth=3  IndexOptions=Index vector (dialog)  Indices=[1 2]  OutputSizes=1
  Sqrt : Sqrt
  Square : Math  Operator=square
  Square1 : Math  Operator=square
  Subtract : Sum  Inputs=+-
  Subtract1 : Sum  Inputs=+-
  Sum : Sum  Inputs=|++
  E : Outport
  wires:
  Constant1/1 -> Demux/1
  Pose/1 -> Selector/1
  Demux/1 -> Subtract/1
  Selector/1 -> Demux1/1
  Demux1/1 -> Subtract/2
  Demux/2 -> Subtract1/1
  Demux1/2 -> Subtract1/2
  Subtract/1 -> Square/1
  Subtract1/1 -> Square1/1
  Square/1 -> Sum/1
  Square1/1 -> Sum/2
  Sum/1 -> Sqrt/1
  Sqrt/1 -> Compare To Constant/1, Scope1/1  "xFinal"
  Compare To Constant/1 -> E/1  "End"

== system sm_amrPioneer3DX_path_follow/Robot/Camera ==
  Reference Frame Camera Left : sm_lib/Frames and Transforms/Reference Frame
  Reference Frame Camera Rear : sm_lib/Frames and Transforms/Reference Frame
  Transform Camera Left : sm_lib/Frames and Transforms/Rigid Transform  RotationMethod=RotationSequence  FollAlignAxisA=+X  BaseAlignAxisA=+Y  FollAlignAxisB=+Y  BaseAlignAxisB=+Z  RotationStandardAxis=+Y  RotationAngle=10  RotationAngleUnits=deg  RotationArbitraryAxis=[0 0 1]  RotationSequenceAxes=FollowerAxes  RotationSequence=ZYX  RotationSequenceAngles=[-90 10 0]  RotationSequenceAnglesUnits=deg  RotationMatrix=[1 0 0; 0 1 0; 0 0 1]  Quaternion=[1 0 0 0]  TranslationMethod=Cartesian  TranslationCartesianOffset=[0 0.6 -0.05]  TranslationCartesianOffsetUnits=m  TranslationStandardAxis=+Z  TranslationStandardOffset=0  TranslationStandardOffsetUnits=m  TranslationROffset=0  TranslationROffsetUnits=m  TranslationThetaOffset=0  TranslationThetaOffsetUnits=deg  TranslationZOffset=0  TranslationZOffsetUnits=m
  Transform Camera Rear : sm_lib/Frames and Transforms/Rigid Transform  RotationMethod=StandardAxis  FollAlignAxisA=+X  BaseAlignAxisA=+Y  FollAlignAxisB=+Y  BaseAlignAxisB=+Z  RotationStandardAxis=+Y  RotationAngle=10  RotationAngleUnits=deg  RotationArbitraryAxis=[0 0 1]  RotationSequenceAxes=FollowerAxes  RotationSequence=XYX  RotationSequenceAngles=[0 0 0]  RotationSequenceAnglesUnits=deg  RotationMatrix=[1 0 0; 0 1 0; 0 0 1]  Quaternion=[1 0 0 0]  TranslationMethod=Cartesian  TranslationCartesianOffset=[-0.8 0 0.2]  TranslationCartesianOffsetUnits=m  TranslationStandardAxis=+Z  TranslationStandardOffset=0  TranslationStandardOffsetUnits=m  TranslationROffset=0  TranslationROffsetUnits=m  TranslationThetaOffset=0  TranslationThetaOffsetUnits=deg  TranslationZOffset=0  TranslationZOffsetUnits=m
  B : PMIOPort  Side=Left
  connections:
  Transform Camera Rear/RConn1 -- Reference Frame Camera Rear/RConn1
  B/RConn1 -- Transform Camera Left/LConn1 -- Transform Camera Rear/LConn1
  Reference Frame Camera Left/RConn1 -- Transform Camera Left/RConn1

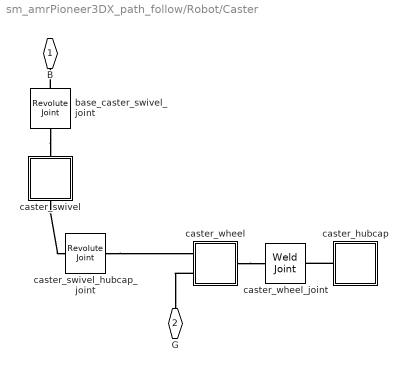
== system sm_amrPioneer3DX_path_follow/Robot/Caster ==
  base_caster_swivel_joint : sm_lib/Joints/Revolute Joint  JointMode=Normal  CompositeWrenchDir=FollowerOnBase  CompositeWrenchFrame=BaseFrame  SenseConstraintForce=off  SenseConstraintTorque=off  SenseTotalForce=off  SenseTotalTorque=off  PositionTargetSpecify=off  PositionTargetPriority=High  PositionTargetValue=0  PositionTargetValueUnits=deg  VelocityTargetSpecify=off  VelocityTargetPriority=High  VelocityTargetValue=0  VelocityTargetValueUnits=deg/s  EquilibriumPosition=0  EquilibriumPositionUnits=deg  SpringStiffness=0  SpringStiffnessUnits=N*m/deg  DampingCoefficient=0  DampingCoefficientUnits=m^2*kg/s/rad  LowerLimitSpecify=off  LowerLimitBound=-90  LowerLimitBoundUnits=deg  LowerLimitStiffness=1e4  LowerLimitStiffnessUnits=N*m/deg  LowerLimitDamping=10  LowerLimitDampingUnits=N*m/(deg/s)  LowerLimitTransitionRegionWidth=0.1  LowerLimitTransitionRegionWidthUnits=deg  UpperLimitSpecify=off  UpperLimitBound=90  UpperLimitBoundUnits=deg  UpperLimitStiffness=1e4  UpperLimitStiffnessUnits=N*m/deg  UpperLimitDamping=10  UpperLimitDampingUnits=N*m/(deg/s)  UpperLimitTransitionRegionWidth=0.1  UpperLimitTransitionRegionWidthUnits=deg  TorqueActuationMode=NoTorque  MotionActuationMode=ComputedMotion  SensePosition=off  SenseVelocity=off  SenseAcceleration=off  SenseTorqueForce=off  SenseLowerLimitTorqueForce=off  SenseUpperLimitTorqueForce=off
  caster_hubcap : Subsystem
  caster_swivel : Subsystem
  caster_swivel_hubcap_joint : sm_lib/Joints/Revolute Joint  JointMode=Normal  CompositeWrenchDir=FollowerOnBase  CompositeWrenchFrame=BaseFrame  SenseConstraintForce=off  SenseConstraintTorque=off  SenseTotalForce=off  SenseTotalTorque=off  PositionTargetSpecify=off  PositionTargetPriority=High  PositionTargetValue=0  PositionTargetValueUnits=deg  VelocityTargetSpecify=off  VelocityTargetPriority=High  VelocityTargetValue=0  VelocityTargetValueUnits=deg/s  EquilibriumPosition=0  EquilibriumPositionUnits=deg  SpringStiffness=0  SpringStiffnessUnits=N*m/deg  DampingCoefficient=0  DampingCoefficientUnits=m^2*kg/s/rad  LowerLimitSpecify=off  LowerLimitBound=-90  LowerLimitBoundUnits=deg  LowerLimitStiffness=1e4  LowerLimitStiffnessUnits=N*m/deg  LowerLimitDamping=10  LowerLimitDampingUnits=N*m/(deg/s)  LowerLimitTransitionRegionWidth=0.1  LowerLimitTransitionRegionWidthUnits=deg  UpperLimitSpecify=off  UpperLimitBound=90  UpperLimitBoundUnits=deg  UpperLimitStiffness=1e4  UpperLimitStiffnessUnits=N*m/deg  UpperLimitDamping=10  UpperLimitDampingUnits=N*m/(deg/s)  UpperLimitTransitionRegionWidth=0.1  UpperLimitTransitionRegionWidthUnits=deg  TorqueActuationMode=NoTorque  MotionActuationMode=ComputedMotion  SensePosition=off  SenseVelocity=off  SenseAcceleration=off  SenseTorqueForce=off  SenseLowerLimitTorqueForce=off  SenseUpperLimitTorqueForce=off
  caster_wheel : Subsystem
  caster_wheel_joint : sm_lib/Joints/Weld Joint  JointMode=Normal  CompositeWrenchDir=FollowerOnBase  CompositeWrenchFrame=BaseFrame  SenseConstraintForce=off  SenseConstraintTorque=off  SenseTotalForce=off  SenseTotalTorque=off
  B : PMIOPort  Side=Left
  G : PMIOPort  Port=2  Side=Right
  connections:
  caster_swivel/RConn1 -- caster_swivel_hubcap_joint/LConn1
  caster_wheel/RConn1 -- caster_wheel_joint/LConn1
  base_caster_swivel_joint/RConn1 -- caster_swivel/LConn1
  base_caster_swivel_joint/LConn1 -- B/RConn1
  caster_hubcap/LConn1 -- caster_wheel_joint/RConn1
  caster_swivel_hubcap_joint/RConn1 -- caster_wheel/LConn1
  caster_wheel/LConn2 -- G/RConn1

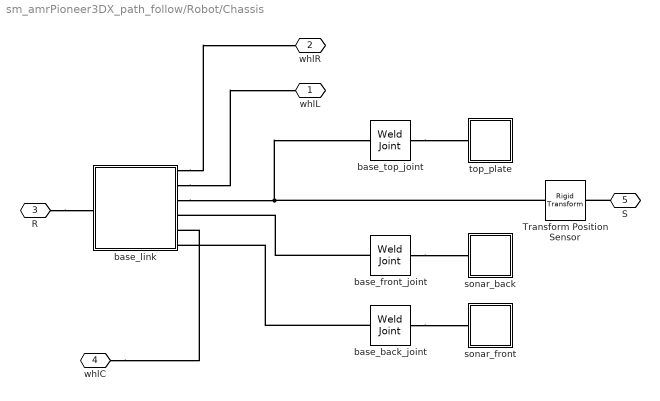
== system sm_amrPioneer3DX_path_follow/Robot/Chassis ==
  Transform Position Sensor : sm_lib/Frames and Transforms/Rigid Transform  RotationMethod=StandardAxis  FollAlignAxisA=+X  BaseAlignAxisA=+Y  FollAlignAxisB=+Y  BaseAlignAxisB=+Z  RotationStandardAxis=+Z  RotationAngle=0  RotationAngleUnits=deg  RotationArbitraryAxis=[0 0 1]  RotationSequenceAxes=FollowerAxes  RotationSequence=XYX  RotationSequenceAngles=[0 0 0]  RotationSequenceAnglesUnits=deg  RotationMatrix=[1 0 0; 0 1 0; 0 0 1]  Quaternion=[1 0 0 0]  TranslationMethod=None  TranslationCartesianOffset=[0 0 0]  TranslationCartesianOffsetUnits=m  TranslationStandardAxis=+Z  TranslationStandardOffset=0  TranslationStandardOffsetUnits=m  TranslationROffset=0  TranslationROffsetUnits=m  TranslationThetaOffset=0  TranslationThetaOffsetUnits=deg  TranslationZOffset=0  TranslationZOffsetUnits=m
  base_back_joint : sm_lib/Joints/Weld Joint  JointMode=Normal  CompositeWrenchDir=FollowerOnBase  CompositeWrenchFrame=BaseFrame  SenseConstraintForce=off  SenseConstraintTorque=off  SenseTotalForce=off  SenseTotalTorque=off
  base_front_joint : sm_lib/Joints/Weld Joint  JointMode=Normal  CompositeWrenchDir=FollowerOnBase  CompositeWrenchFrame=BaseFrame  SenseConstraintForce=off  SenseConstraintTorque=off  SenseTotalForce=off  SenseTotalTorque=off
  base_link : Subsystem
  base_top_joint : sm_lib/Joints/Weld Joint  JointMode=Normal  CompositeWrenchDir=FollowerOnBase  CompositeWrenchFrame=BaseFrame  SenseConstraintForce=off  SenseConstraintTorque=off  SenseTotalForce=off  SenseTotalTorque=off
  sonar_back : Subsystem
  sonar_front : Subsystem
  top_plate : Subsystem
  whlL : PMIOPort  Side=Right
  whlR : PMIOPort  Port=2  Side=Right
  R : PMIOPort  Port=3  Side=Left
  whlC : PMIOPort  Port=4  Side=Left
  S : PMIOPort  Port=5  Side=Left
  connections:
  base_back_joint/LConn1 -- base_link/RConn6
  base_back_joint/RConn1 -- sonar_front/LConn1
  base_link/RConn3 -- Transform Position Sensor/LConn1 -- base_top_joint/LConn1
  base_front_joint/RConn1 -- sonar_back/LConn1
  base_front_joint/LConn1 -- base_link/RConn4
  whlC/RConn1 -- base_link/RConn5
  base_top_joint/RConn1 -- top_plate/LConn1
  base_link/RConn2 -- whlL/RConn1
  R/RConn1 -- base_link/LConn1
  base_link/RConn1 -- whlR/RConn1
  S/RConn1 -- Transform Position Sensor/RConn1

== system sm_amrPioneer3DX_path_follow/Robot/Path ==
  Extruded Solid Path : sm_lib/Body Elements/Extruded Solid  ExtrusionType=General  PolygonNumSides=3  PolygonOuterRadius=1  PolygonOuterRadiusUnits=m  ExportEntireGeometry=off  ExtrusionCrossSection=xy_data  ExtrusionCrossSectionUnits=m  ExportConvexHullGeometry=off  ExtrusionLength=path_depth  ExtrusionLengthUnits=m  InertiaType=CalculateFromGeometry  BasedOnType=Density  Density=1000  DensityUnits=kg/m^3  Mass=1  MassUnits=kg  CenterOfMass=[0 0 0]  CenterOfMassUnits=m  MomentsOfInertia=[1 1 1]  MomentsOfInertiaUnits=kg*m^2  ProductsOfInertia=[0 0 0]  ProductsOfInertiaUnits=kg*m^2  GraphicType=FromGeometry  MarkerShape=Sphere  MarkerSize=10  GraphicVisPropType=SimpleVisualProperties  GraphicDiffuseColor=clr_path  GraphicOpacity=opc_path  GraphicSpecularColor=[0.5 0.5 0.5 1.0]  GraphicAmbientColor=[0.15 0.15 0.15 1.0]  GraphicEmissiveColor=[0.0 0.0 0.0 1.0]  GraphicShininess=75  DoExposeReferenceFrame=on  SerializedFrames=<Frames/>
  Point Cloud Waypoints : sm_lib/Curves and Surfaces/Point Cloud  CoordinatesMatrix=[waypoint_list zeros(size(waypoint_list,1),1)]  CoordinatesMatrixUnits=m  GraphicType=MarkerCloud  GraphicSphereRadius=pt_rad  GraphicSphereRadiusUnits=m  GraphicVisPropType=SimpleVisualProperties  GraphicDiffuseColor=pt_clr  GraphicOpacity=pt_opc  GraphicSpecularColor=[0.5 0.5 0.5 1.0]  GraphicAmbientColor=[0.15 0.15 0.15 1.0]  GraphicEmissiveColor=[0.0 0.0 0.0 1.0]  GraphicShininess=75
  Transform Upper Surface : sm_lib/Frames and Transforms/Rigid Transform  RotationMethod=None  FollAlignAxisA=+X  BaseAlignAxisA=+Y  FollAlignAxisB=+Y  BaseAlignAxisB=+Z  RotationStandardAxis=+Z  RotationAngle=0.0  RotationAngleUnits=deg  RotationArbitraryAxis=[0 0 1]  RotationSequenceAxes=FollowerAxes  RotationSequence=XYX  RotationSequenceAngles=[0 0 0]  RotationSequenceAnglesUnits=deg  RotationMatrix=[1 0 0; 0 1 0; 0 0 1]  Quaternion=[1 0 0 0]  TranslationMethod=StandardAxis  TranslationCartesianOffset=[0 0 0]  TranslationCartesianOffsetUnits=m  TranslationStandardAxis=+Z  TranslationStandardOffset=-path_depth/2  TranslationStandardOffsetUnits=m  TranslationROffset=0  TranslationROffsetUnits=m  TranslationThetaOffset=0  TranslationThetaOffsetUnits=deg  TranslationZOffset=0  TranslationZOffsetUnits=m
  W : PMIOPort  Side=Left
  connections:
  Transform Upper Surface/RConn1 -- Extruded Solid Path/RConn1 -- Point Cloud Waypoints/LConn1
  W/RConn1 -- Transform Upper Surface/LConn1

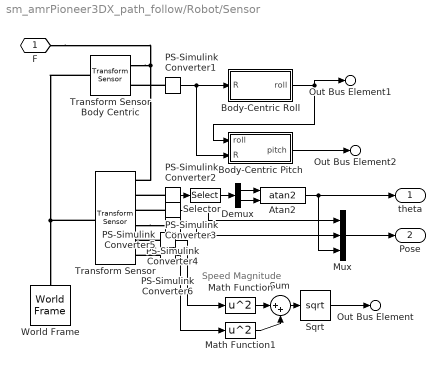
== system sm_amrPioneer3DX_path_follow/Robot/Sensor ==
  note: Speed Magnitude
  Atan2 : Trigonometry  Operator=atan2
  Body-Centric Pitch : Subsystem
  Body-Centric Roll : Subsystem
  Demux : Demux  Outputs=2
  Math Function : Math  Operator=square
  Math Function1 : Math  Operator=square
  Mux : Mux  Inputs=3
  PS-Simulink Converter{1..6} (6 alike) : nesl_utility/PS-Simulink Converter  PhysicalDomain=network_engine_domain  SubClassName=ps_output  LeftPortType=input  RightPortType=output  PseudoPeriodic=off  Frequencies=[]  VectorFormat=1-D array  Unit=inherit  AffineConversion=off
  Selector : Selector  NumberOfDimensions=2  InputPortWidth=3  IndexOptions=Index vector (dialog),Index vector (dialog)  Indices=[2,1],1  OutputSizes=1,1
  Sqrt : Sqrt
  Sum : Sum  Inputs=|++
  Transform Sensor : sm_lib/Frames and Transforms/Transform Sensor  MeasurementFrame=World  RotationSequence=XYX  SenseAngle=off  SenseAxis=off  SenseQ=off  SenseR=on  SenseRotationSequence=off  SenseOmegaX=off  SenseOmegaY=off  SenseOmegaZ=off  SenseOmega=off  SenseQDot=off  SenseRDot=off  SenseRotationSequenceDot=off  SenseAlphaX=off  SenseAlphaY=off  SenseAlphaZ=off  SenseAlpha=off  SenseQDDot=off  SenseRDDot=off  SenseX=on  SenseY=on  SenseZ=off  SenseXYZ=off  SenseRad=off  SenseAzim=off  SenseDist=off  SenseInc=off  SenseXDot=on  SenseYDot=on  SenseZDot=off  SenseXYZDot=off  SenseRadDot=off  SenseAzimDot=off  SenseDistDot=off  SenseIncDot=off  SenseXDDot=off  SenseYDDot=off  SenseZDDot=off  SenseXYZDDot=off  SenseRadDDot=off  SenseAzimDDot=off  SenseDistDDot=off  SenseIncDDot=off
  Transform Sensor Body Centric : sm_lib/Frames and Transforms/Transform Sensor  MeasurementFrame=World  RotationSequence=XYX  SenseAngle=off  SenseAxis=off  SenseQ=off  SenseR=on  SenseRotationSequence=off  SenseOmegaX=off  SenseOmegaY=off  SenseOmegaZ=off  SenseOmega=off  SenseQDot=off  SenseRDot=off  SenseRotationSequenceDot=off  SenseAlphaX=off  SenseAlphaY=off  SenseAlphaZ=off  SenseAlpha=off  SenseQDDot=off  SenseRDDot=off  SenseX=off  SenseY=off  SenseZ=off  SenseXYZ=off  SenseRad=off  SenseAzim=off  SenseDist=off  SenseInc=off  SenseXDot=off  SenseYDot=off  SenseZDot=off  SenseXYZDot=off  SenseRadDot=off  SenseAzimDot=off  SenseDistDot=off  SenseIncDot=off  SenseXDDot=off  SenseYDDot=off  SenseZDDot=off  SenseXYZDDot=off  SenseRadDDot=off  SenseAzimDDot=off  SenseDistDDot=off  SenseIncDDot=off
  World Frame : sm_lib/Frames and Transforms/World Frame
  F : PMIOPort  Side=Left
  theta : Outport
  Pose : Outport  Port=2
  Out Bus Element : Outport  Port=3  PortName=Body  Element=v
  Out Bus Element1 : Outport  Port=3  PortName=Body  Element=roll
  Out Bus Element2 : Outport  Port=3  PortName=Body  Element=pitch
  wires:
  Demux/2 -> Atan2/2
  Math Function1/1 -> Sum/2
  Math Function/1 -> Sum/1
  Atan2/1 -> theta/1, Mux/3
  PS-Simulink Converter4/1 -> Mux/2
  PS-Simulink Converter3/1 -> Mux/1
  Sum/1 -> Sqrt/1
  Selector/1 -> Demux/1
  PS-Simulink Converter2/1 -> Selector/1
  Mux/1 -> Pose/1
  PS-Simulink Converter6/1 -> Math Function1/1
  Demux/1 -> Atan2/1
  PS-Simulink Converter5/1 -> Math Function/1
  Sqrt/1 -> Out Bus Element/1
  PS-Simulink Converter1/1 -> Body-Centric Pitch/2(R), Body-Centric Roll/1(R)
  Body-Centric Roll/1(roll) -> Out Bus Element1/1, Body-Centric Pitch/1(roll)
  Body-Centric Pitch/1(pitch) -> Out Bus Element2/1
  connections:
  PS-Simulink Converter6/LConn1 -- Transform Sensor/RConn6
  PS-Simulink Converter2/LConn1 -- Transform Sensor/RConn2
  PS-Simulink Converter5/LConn1 -- Transform Sensor/RConn5
  Transform Sensor/RConn4 -- PS-Simulink Converter4/LConn1
  F/RConn1 -- Transform Sensor/RConn1 -- Transform Sensor Body Centric/RConn1
  PS-Simulink Converter3/LConn1 -- Transform Sensor/RConn3
  Transform Sensor/LConn1 -- World Frame/RConn1 -- Transform Sensor Body Centric/LConn1
  PS-Simulink Converter1/LConn1 -- Transform Sensor Body Centric/RConn2

== system sm_amrPioneer3DX_path_follow/Robot/Wheel L ==
  left_hub : Subsystem
  left_wheel : Subsystem
  left_wheel_joint : sm_lib/Joints/Weld Joint  JointMode=Normal  CompositeWrenchDir=FollowerOnBase  CompositeWrenchFrame=BaseFrame  SenseConstraintForce=off  SenseConstraintTorque=off  SenseTotalForce=off  SenseTotalTorque=off
  F : PMIOPort  Side=Right
  G : PMIOPort  Port=2  Side=Left
  connections:
  left_wheel/LConn1 -- left_wheel_joint/RConn1
  left_hub/RConn1 -- left_wheel_joint/LConn1
  left_wheel/LConn2 -- G/RConn1
  left_hub/LConn1 -- F/RConn1

== system sm_amrPioneer3DX_path_follow/Robot/WheelR ==
  right_hub : Subsystem
  right_wheel : Subsystem
  right_wheel_joint : sm_lib/Joints/Weld Joint  JointMode=Normal  CompositeWrenchDir=FollowerOnBase  CompositeWrenchFrame=BaseFrame  SenseConstraintForce=off  SenseConstraintTorque=off  SenseTotalForce=off  SenseTotalTorque=off
  F : PMIOPort  Side=Left
  G : PMIOPort  Port=2  Side=Right
  connections:
  right_wheel/LConn1 -- right_wheel_joint/RConn1
  right_hub/RConn1 -- right_wheel_joint/LConn1
  right_wheel/LConn2 -- G/RConn1
  right_hub/LConn1 -- F/RConn1

== system sm_amrPioneer3DX_path_follow/Robot/Caster/caster_hubcap ==
  Inertia : sm_lib/Body Elements/Inertia  InertiaType=Custom  Mass=0.01  MassUnits=kg  CenterOfMass=[0, 0, 0]  CenterOfMassUnits=m  MomentsOfInertia=[0.012411765597, 0.015218160428, 0.011763977943]  MomentsOfInertiaUnits=kg*m^2  ProductsOfInertia=[-4.273467e-06, 0.00050272983, -0.000711733678]  ProductsOfInertiaUnits=kg*m^2  GraphicType=None  MarkerShape=Inertia  MarkerSize=20  GraphicVisPropType=SimpleVisualProperties  GraphicDiffuseColor=[0.5 0.5 0.5]  GraphicOpacity=1.0  GraphicSpecularColor=[0.5 0.5 0.5 1.0]  GraphicAmbientColor=[0.15 0.15 0.15 1.0]  GraphicEmissiveColor=[0.0 0.0 0.0 1.0]  GraphicShininess=75
  InertiaOriginTransform : sm_lib/Frames and Transforms/Rigid Transform  RotationMethod=RotationSequence  FollAlignAxisA=+X  BaseAlignAxisA=+Y  FollAlignAxisB=+Y  BaseAlignAxisB=+Z  RotationStandardAxis=+Z  RotationAngle=0.0  RotationAngleUnits=deg  RotationArbitraryAxis=[0 0 1]  RotationSequenceAxes=BaseAxes  RotationSequence=XYZ  RotationSequenceAngles=[0, 0, 0]  RotationSequenceAnglesUnits=rad  RotationMatrix=[1 0 0; 0 1 0; 0 0 1]  Quaternion=[1 0 0 0]  TranslationMethod=Cartesian  TranslationCartesianOffset=[0, 0, 0]  TranslationCartesianOffsetUnits=m  TranslationStandardAxis=+Z  TranslationStandardOffset=0  TranslationStandardOffsetUnits=m  TranslationROffset=0  TranslationROffsetUnits=m  TranslationThetaOffset=0  TranslationThetaOffsetUnits=deg  TranslationZOffset=0  TranslationZOffsetUnits=m
  ReferenceFrame : sm_lib/Frames and Transforms/Reference Frame
  Visual : sm_lib/Body Elements/File Solid  ExtGeomFileName=amr3dx_caster_hubcap.stl  UnitType=Custom  ExtGeomFileUnits=m  StepReaderType=HEX  ExportConvexHullGeometry=off  InertiaType=Custom  BasedOnType=DensityFromFile  Density=1000  DensityUnits=kg/m^3  Mass=0  MassUnits=kg  CenterOfMass=[0, 0, 0]  CenterOfMassUnits=m  MomentsOfInertia=[0, 0, 0]  MomentsOfInertiaUnits=kg*m^2  ProductsOfInertia=[0, 0, 0]  ProductsOfInertiaUnits=kg*m^2  GraphicType=FromGeometry  MarkerShape=Sphere  MarkerSize=10  GraphicVisPropType=SimpleVisualProperties  GraphicDiffuseColor=[0.5, 0.5, 0.5]  GraphicOpacity=1  GraphicSpecularColor=[0.5 0.5 0.5 1.0]  GraphicAmbientColor=[0.15 0.15 0.15 1.0]  GraphicEmissiveColor=[0.0 0.0 0.0 1.0]  GraphicShininess=75  DoExposeReferenceFrame=on  SerializedFrames=<Frames/>
  VisualOriginTransform : sm_lib/Frames and Transforms/Rigid Transform  RotationMethod=RotationSequence  FollAlignAxisA=+X  BaseAlignAxisA=+Y  FollAlignAxisB=+Y  BaseAlignAxisB=+Z  RotationStandardAxis=+Z  RotationAngle=0.0  RotationAngleUnits=deg  RotationArbitraryAxis=[0 0 1]  RotationSequenceAxes=BaseAxes  RotationSequence=XYZ  RotationSequenceAngles=[0, 0, 0]  RotationSequenceAnglesUnits=rad  RotationMatrix=[1 0 0; 0 1 0; 0 0 1]  Quaternion=[1 0 0 0]  TranslationMethod=Cartesian  TranslationCartesianOffset=[0, 0, 0]  TranslationCartesianOffsetUnits=m  TranslationStandardAxis=+Z  TranslationStandardOffset=0  TranslationStandardOffsetUnits=m  TranslationROffset=0  TranslationROffsetUnits=m  TranslationThetaOffset=0  TranslationThetaOffsetUnits=deg  TranslationZOffset=0  TranslationZOffsetUnits=m
  F : PMIOPort  Side=Left
  connections:
  Inertia/RConn1 -- InertiaOriginTransform/RConn1
  InertiaOriginTransform/LConn1 -- ReferenceFrame/RConn1 -- F/RConn1 -- VisualOriginTransform/LConn1
  Visual/RConn1 -- VisualOriginTransform/RConn1
